simulink model "HA_sim"  (R2022a)
settings: Solver=ode45  StartTime=0.0  StopTime=10  RelTol=1e-3  EnableMultiTasking=on
InitFcn:
  | HA_Control_Design;
values from neighbouring files (symbols this model uses):
  A = [0 0 1 0;      0 0 0 1;      (3*M*g*L + 6*m*g*l)/(2*M*L^2+6*m*l^2) 0 0 0;      -(3*M*g*L + 6*m*g*l)/(2*M*L^2+6*m*l^2) 0 0 0;      ]    [HA_Control_Design.m]
  B = [0 ; 0 ; -6/(2*M*L^2+6*m*l^2); (6*J + 2*M*L^2 + 6*m*l^2)/(J*(2*M*L^2 + 6*m*l^2))]    [HA_Control_Design.m]
  g = 9.81    [HA_Control_Design.m]
  J = 10.4    [HA_Control_Design.m]
  K = lqr(A,B,Q,R)    [HA_Control_Design.m]
  L = 2    [HA_Control_Design.m]
  l = 1.5    [HA_Control_Design.m]
  M = 75    [HA_Control_Design.m]
  m = 5    [HA_Control_Design.m]
  psi0 = 0    [HA_Control_Design.m]
  psidot0 = 0    [HA_Control_Design.m]
  theta0 = 0.1    [HA_Control_Design.m]
  thetadot0 = 0    [HA_Control_Design.m]
  x0 = [theta0; psi0; thetadot0; psidot0]    [HA_Control_Design.m]    (also in sfun_keyboard_input_v1_01.m = 43)
libraries: vrlib x5, aerolibanimutils x1
Description:
  | Simulink(R) 3D Animation(TM) - Tutorial #3
  | 
  | Tutorial model to be used for 3D World Editor authoring example in the documentation.
  | After creating the virtual world according to the instructions in the documentation, include the VR block
  | in the model and connect B1, B2 coordinates and S scaling to corresponding nodes in
  | the virtual world.
settings Model: ExtModeTrigMode=oneshot  ExtModeArmWhenConnect=off  Creator=The MathWorks, Inc.  LastModifiedBy=vcichella
settings SolverCC: AlgebraicLoopSolver=TrustRegion
settings DataIOCC: LimitDataPoints=on  SaveFormat=Array  SaveOutput=off  SaveTime=off  ReturnWorkspaceOutputs=off  SignalLoggingName=logsOut
settings OptimizationCC: BooleanDataType=off  ExpressionDepthLimit=2147483647  InitFltsAndDblsToZero=on  LifeSpan=inf
settings DebuggingCC: UnderspecifiedInitializationDetection=Classic  MergeDetectMultiDrivingBlocksExec=none  CheckExecutionContextPreStartOutputMsg=on  SignalResolutionControl=TryResolveAllWithWarning  MultiTaskDSMMsg=warning  MultiTaskCondExecSysMsg=none  FcnCallInpInsideContextMsg=warning  UnconnectedInputMsg=warning  UnconnectedOutputMsg=warning  UnconnectedLineMsg=warning  StateNameClashWarn=warning  SymbolicDimsDataTypeCodeGenerationDiagnostic=none  SFUnexpectedBacktrackingDiag=warning  SFNoUnconditionalDefaultTransitionDiag=warning  SFExecutionAtInitializationDiag=none  SFMachineParentedDataDiag=warning  ArithmeticOperatorsInVariantConditions=warning
settings HardwareCC: ProdBitPerPointer=32  ProdBitPerSizeT=32  ProdBitPerPtrDiffT=32  ProdLargestAtomicFloat=None  ProdIntDivRoundTo=Undefined  ProdEndianess=Unspecified  ProdWordSize=32  ProdHWDeviceType=32-bit Generic  TargetUnknown=on
settings ModelReferenceCC: UpdateModelReferenceTargets=IfOutOfDate  PropagateSignalLabelsOutOfModel=off
settings SFSimCC: SimUseLocalCustomCode=off  CustomCodeUndefinedFunction=UseInterfaceOnly
settings RTWCC: RTWUseLocalCustomCode=off
settings CodeAppCC: StateflowObjectComments=on
settings GRTTargetCC: TargetFcnLib=ansi_tfl_tmw.mat  TargetLangStandard=C89/C90 (ANSI)  CombineOutputUpdateFcns=off  GRTInterface=on
settings ConfigComp: CovMetricSettings=d  CovSaveCumulativeToWorkspaceVar=on  CovSaveSingleToWorkspaceVar=on  CovExternalEMLEnable=off  CovSFcnEnable=off

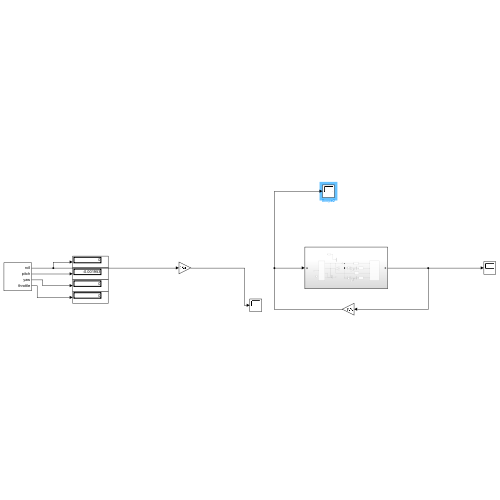
[thumbnail: Simulink's stored preview of the top-level diagram]
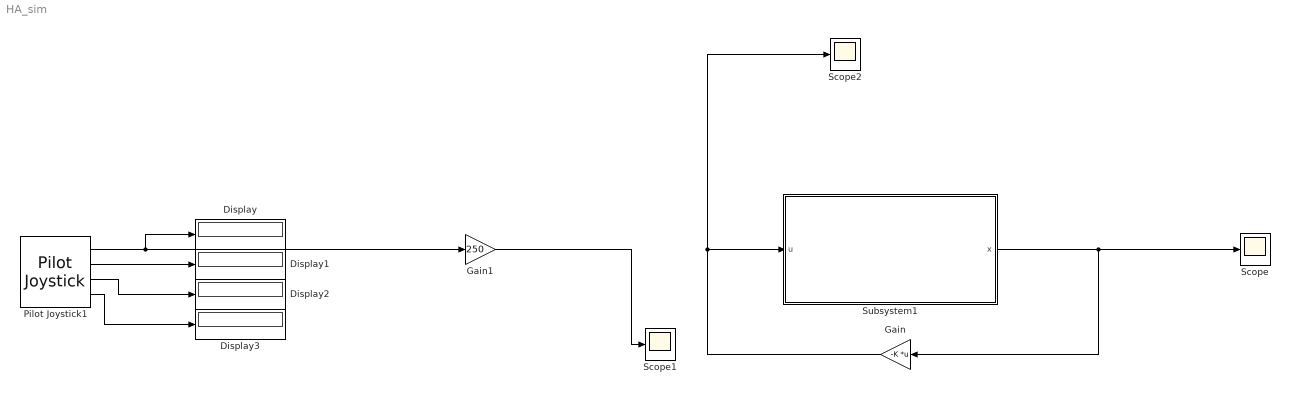
== system HA_sim ==
  Display{,1..3} (4 alike) : Display
  Gain : Gain  Gain=-K  Multiplication=Matrix(K*u)
  Gain1 : Gain  Gain=250
  Pilot Joystick1 : aerolibanimutils/Pilot Joystick  JoystickID=Joystick1  OutputConfiguration=FourAxis  SampleTime=1/30
  Scope : Scope
  Scope1 : Scope
  Scope2 : Scope
  Subsystem1 : Subsystem
  wires:
  Pilot Joystick1/1 -> Display/1, Gain1/1
  Subsystem1/1(x) -> Gain/1, Scope/1
  Pilot Joystick1/2 -> Display1/1
  Pilot Joystick1/3 -> Display2/1
  Pilot Joystick1/4 -> Display3/1
  Gain1/1 -> Scope1/1
  Gain/1 -> Scope2/1, Subsystem1/1(u)

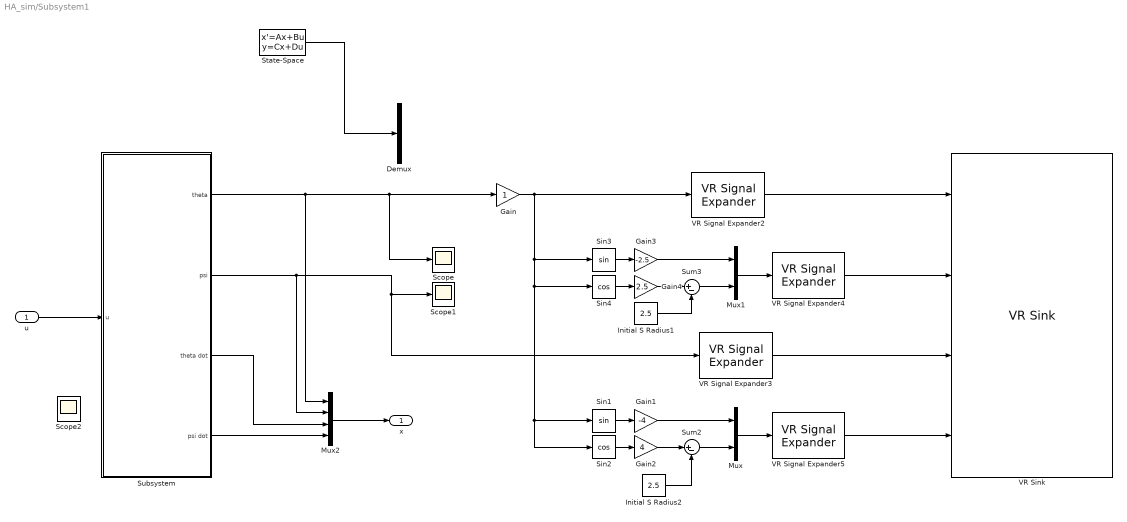
== system HA_sim/Subsystem1 ==
  u : Inport
  Demux : Demux
  Gain : Gain
  Gain1 : Gain  Gain=-4
  Gain2 : Gain  Gain=4
  Gain3 : Gain  Gain=-2.5
  Gain4 : Gain  Gain=2.5
  Initial S Radius1 : Constant  Value=2.5
  Initial S Radius2 : Constant  Value=2.5
  Mux : Mux  Inputs=2
  Mux1 : Mux  Inputs=2
  Mux2 : Mux
  Scope : Scope
  Scope1 : Scope
  Scope2 : Scope
  Sin1 : Trigonometry
  Sin2 : Trigonometry  Operator=cos
  Sin3 : Trigonometry
  Sin4 : Trigonometry  Operator=cos
  State-Space : StateSpace  A=A  B=B  C=eye(4)  D=zeros(4,1)  InitialCondition=x0
  Subsystem : Subsystem
  Sum2 : Sum  Inputs=|+-  InputSameDT=on  SaturateOnIntegerOverflow=on  OutDataTypeStr=Inherit: Same as first input
  Sum3 : Sum  Inputs=|+-  InputSameDT=on  SaturateOnIntegerOverflow=on  OutDataTypeStr=Inherit: Same as first input
  VR Signal Expander2 : vrlib/VR Signal Expander  outwidth=4  outidx=4
  VR Signal Expander3 : vrlib/VR Signal Expander  outwidth=4  outidx=4
  VR Signal Expander4 : vrlib/VR Signal Expander  outwidth=3  outidx=[1 2]
  VR Signal Expander5 : vrlib/VR Signal Expander  outwidth=3  outidx=[1 2]
  VR Sink : vrlib/VR Sink  InstantiateOnLoad=on  SampleTime=0.1  ViewEnable=on  RemoteChange=off  RemoteView=off  FieldsWritten=B1.rotation.4.1.1.double#B1.translation.3.1.1.double#B2.rotation.4.1.1.double#B2.translation.3.1.1.double  WorldFileName=vr_highwire.x3d  WorldDescription=vr_highwire  AutoView=on  VideoDimensions=[]  AllowVariableSize=off
  x : Outport
  wires:
  VR Signal Expander5/1 -> VR Sink/4
  Initial S Radius2/1 -> Sum2/2
  Subsystem/2(psi) -> Mux2/2, Scope1/1, VR Signal Expander3/1
  Sin2/1 -> Gain2/1
  Gain2/1 -> Sum2/1
  Subsystem/1(theta) -> Mux2/1, Gain/1, Scope/1
  Mux/1 -> VR Signal Expander5/1
  Gain1/1 -> Mux/1
  Sin4/1 -> Gain4/1
  Sin3/1 -> Gain3/1
  Sum2/1 -> Mux/2
  Mux1/1 -> VR Signal Expander4/1
  Initial S Radius1/1 -> Sum3/2
  VR Signal Expander2/1 -> VR Sink/1
  Sin1/1 -> Gain1/1
  Gain4/1 -> Sum3/1
  Sum3/1 -> Mux1/2
  Gain3/1 -> Mux1/1
  VR Signal Expander4/1 -> VR Sink/2
  VR Signal Expander3/1 -> VR Sink/3
  Subsystem/3(theta dot) -> Mux2/3
  Subsystem/4(psi dot) -> Mux2/4
  State-Space/1 -> Demux/1
  Gain/1 -> Sin3/1, Sin4/1, Sin2/1, Sin1/1, VR Signal Expander2/1
  u/1 -> Subsystem/1(u)
  Mux2/1 -> x/1

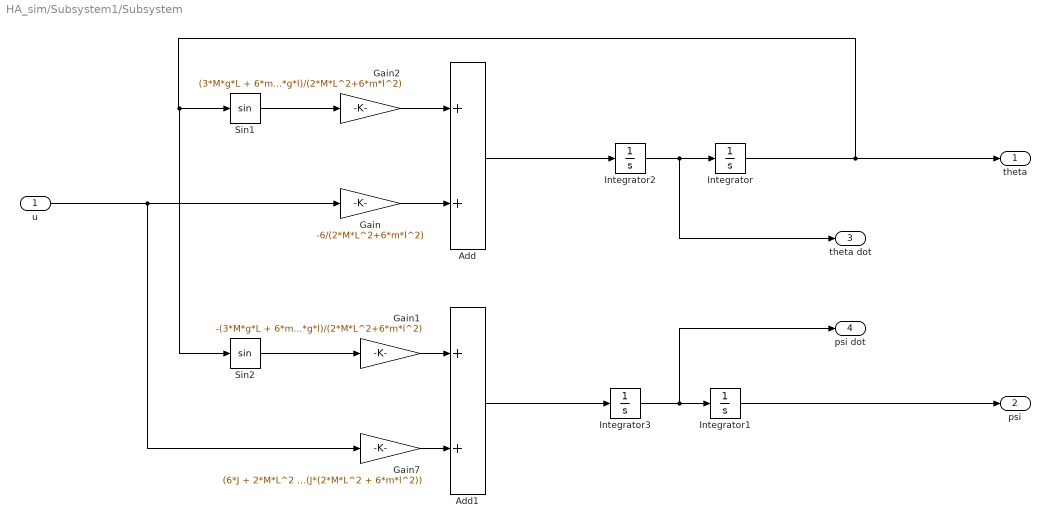
== system HA_sim/Subsystem1/Subsystem ==
  u : Inport
  Add : Sum
  Add1 : Sum
  Gain : Gain  Gain=-6/(2*M*L^2+6*m*l^2)
  Gain1 : Gain  Gain=-(3*M*g*L + 6*m*g*l)/(2*M*L^2+6*m*l^2)
  Gain2 : Gain  Gain=(3*M*g*L + 6*m*g*l)/(2*M*L^2+6*m*l^2)
  Gain7 : Gain  Gain=(6*J + 2*M*L^2 + 6*m*l^2)/(J*(2*M*L^2 + 6*m*l^2))
  Integrator : Integrator  InitialCondition=theta0
  Integrator1 : Integrator  InitialCondition=psi0
  Integrator2 : Integrator  InitialCondition=thetadot0
  Integrator3 : Integrator  InitialCondition=psidot0
  Sin1 : Trigonometry
  Sin2 : Trigonometry
  theta : Outport
  psi : Outport  Port=2
  theta dot : Outport  Port=3
  psi dot : Outport  Port=4
  wires:
  Integrator3/1 -> psi dot/1, Integrator1/1
  Integrator1/1 -> psi/1
  Integrator2/1 -> theta dot/1, Integrator/1
  Gain/1 -> Add/2
  Add/1 -> Integrator2/1
  Integrator/1 -> Sin1/1, Sin2/1, theta/1
  Gain2/1 -> Add/1
  Add1/1 -> Integrator3/1
  u/1 -> Gain7/1, Gain/1
  Gain1/1 -> Add1/1
  Gain7/1 -> Add1/2
  Sin2/1 -> Gain1/1
  Sin1/1 -> Gain2/1
